simulink library "lib_TerCtrl_MASmsg"  (R2026a)
settings: Solver=VariableStepAuto
undefined symbols (not defined in the file): buses_lf, DiscIntNeverNeededParam, entity, iPs_lf, iQs_lf, last_send, m, Ps_lf, Qs_lf, Sb, set_asked, set_DG_up, set_extra_satur, set_sending_cost, v_buses_mod
libraries: simulink x581, sl_discontinuities x14, eeGeneralControl x7
(part 14 of 17)

== system lib_TerCtrl_MASmsg/MAS messages/ID6/Send to neighbor/four ==
  Message : Inport
  Cast1 : EntityMulticast  InputPortMessageModes=m  MulticastTag=ID1
  Cast1all : EntityMulticast  InputPortMessageModes=m  MulticastTag=ID1
  Cast2 : EntityMulticast  InputPortMessageModes=m  MulticastTag=ID3
  Cast2all : EntityMulticast  InputPortMessageModes=m  MulticastTag=ID3
  Cast3 : EntityMulticast  InputPortMessageModes=m  MulticastTag=ID0
  Cast3all : EntityMulticast  InputPortMessageModes=m  MulticastTag=ID0
  Cast4 : EntityMulticast  InputPortMessageModes=m  MulticastTag=ID0
  Cast4all : EntityMulticast  InputPortMessageModes=m  MulticastTag=ID0
  Entity Output Switch : EntityOutputSwitch  InputPortMessageModes=m  OutputPortMessageModes=m,m,m,m,m  NumberOutputPorts=5  SwitchingCriterion=From attribute  SwitchAttributeName=Select  InitialPortSelection=3
      settings: OutputPortMap=o0,o1,o2,o3,o4
  Entity Replicator1 : EntityReplicator  InputPortMessageModes=m  OutputPortMessageModes=m,m,m,m  NumberReplicas=3
      settings: OutputPortMap=o0,o1,o2,o3
  Entity Server : EntityServer  InputPortMessageModes=m  OutputPortMessageModes=m  Capacity=1  ServiceTimeValue=0  EntryAction=entity.Select = select(entity.Dest);
  select : Subsystem  TreatAsAtomicUnit=on
  wires:
  Entity Replicator1/3 -> Cast3all/1
  Entity Replicator1/4 -> Cast4all/1
  Entity Output Switch/5 -> Entity Replicator1/1
  Entity Output Switch/3 -> Cast3/1
  Entity Output Switch/1 -> Cast1/1
  Entity Replicator1/1 -> Cast1all/1
  Entity Replicator1/2 -> Cast2all/1
  Entity Output Switch/2 -> Cast2/1
  Entity Output Switch/4 -> Cast4/1
  Message/1 -> Entity Server/1  "Message"
  Entity Server/1 -> Entity Output Switch/1

== system lib_TerCtrl_MASmsg/MAS messages/ID6/Send to neighbor/one ==
  Message : Inport
  Cast : EntityMulticast  InputPortMessageModes=m  MulticastTag=ID2
  Castall : EntityMulticast  InputPortMessageModes=m  MulticastTag=ID2
  Entity Output Switch1 : EntityOutputSwitch  InputPortMessageModes=m  OutputPortMessageModes=m,m  SwitchingCriterion=From attribute  SwitchAttributeName=Select  InitialPortSelection=3
  Entity Server : EntityServer  InputPortMessageModes=m  OutputPortMessageModes=m  Capacity=1  ServiceTimeValue=0  EntryAction=entity.Select = select(entity.Dest);
  select : Subsystem  TreatAsAtomicUnit=on
  wires:
  Entity Output Switch1/2 -> Castall/1
  Entity Output Switch1/1 -> Cast/1
  Entity Server/1 -> Entity Output Switch1/1
  Message/1 -> Entity Server/1  "Message"

== system lib_TerCtrl_MASmsg/MAS messages/ID6/Send to neighbor/three ==
  Message : Inport
  Cast1 : EntityMulticast  InputPortMessageModes=m  MulticastTag=ID0
  Cast1all : EntityMulticast  InputPortMessageModes=m  MulticastTag=ID0
  Cast2 : EntityMulticast  InputPortMessageModes=m  MulticastTag=ID0
  Cast2all : EntityMulticast  InputPortMessageModes=m  MulticastTag=ID0
  Cast3 : EntityMulticast  InputPortMessageModes=m  MulticastTag=ID0
  Cast3all : EntityMulticast  InputPortMessageModes=m  MulticastTag=ID0
  Entity Output Switch : EntityOutputSwitch  InputPortMessageModes=m  OutputPortMessageModes=m,m,m,m  NumberOutputPorts=4  SwitchingCriterion=From attribute  SwitchAttributeName=Select  InitialPortSelection=3
      settings: OutputPortMap=o0,o1,o2,o3
  Entity Replicator1 : EntityReplicator  InputPortMessageModes=m  OutputPortMessageModes=m,m,m  NumberReplicas=2
      settings: OutputPortMap=o0,o1,o2
  Entity Server : EntityServer  InputPortMessageModes=m  OutputPortMessageModes=m  Capacity=1  ServiceTimeValue=0  EntryAction=entity.Select = select(entity.Dest);
  select : Subsystem  TreatAsAtomicUnit=on
  wires:
  Entity Output Switch/4 -> Entity Replicator1/1
  Entity Output Switch/2 -> Cast2/1
  Entity Replicator1/2 -> Cast2all/1
  Entity Replicator1/1 -> Cast1all/1
  Entity Output Switch/1 -> Cast1/1
  Entity Replicator1/3 -> Cast3all/1
  Entity Output Switch/3 -> Cast3/1
  Message/1 -> Entity Server/1  "Message"
  Entity Server/1 -> Entity Output Switch/1

== system lib_TerCtrl_MASmsg/MAS messages/ID6/Send to neighbor/two ==
  Message : Inport
  Cast1 : EntityMulticast  InputPortMessageModes=m  MulticastTag=ID5
  Cast1all : EntityMulticast  InputPortMessageModes=m  MulticastTag=ID5
  Cast2 : EntityMulticast  InputPortMessageModes=m  MulticastTag=ID7
  Cast2all : EntityMulticast  InputPortMessageModes=m  MulticastTag=ID7
  Entity Output Switch : EntityOutputSwitch  InputPortMessageModes=m  OutputPortMessageModes=m,m,m  NumberOutputPorts=3  SwitchingCriterion=From attribute  SwitchAttributeName=Select  InitialPortSelection=3
      settings: OutputPortMap=o0,o1,o2
  Entity Replicator1 : EntityReplicator  InputPortMessageModes=m  OutputPortMessageModes=m,m
  Entity Server : EntityServer  InputPortMessageModes=m  OutputPortMessageModes=m  Capacity=1  ServiceTimeValue=0  EntryAction=entity.Select = select(entity.Dest);
  select : Subsystem  TreatAsAtomicUnit=on
  wires:
  Entity Output Switch/3 -> Entity Replicator1/1
  Entity Replicator1/2 -> Cast2all/1
  Entity Replicator1/1 -> Cast1all/1
  Message/1 -> Entity Server/1  "Message"
  Entity Output Switch/1 -> Cast1/1
  Entity Output Switch/2 -> Cast2/1
  Entity Server/1 -> Entity Output Switch/1

== system lib_TerCtrl_MASmsg/MAS messages/ID6/Send to neighbor1/five ==
  Message : Inport
  Cast1 : EntityMulticast  InputPortMessageModes=m  MulticastTag=ID2
  Cast1all : EntityMulticast  InputPortMessageModes=m  MulticastTag=ID2
  Cast2 : EntityMulticast  InputPortMessageModes=m  MulticastTag=ID2
  Cast2all : EntityMulticast  InputPortMessageModes=m  MulticastTag=ID2
  Cast3 : EntityMulticast  InputPortMessageModes=m  MulticastTag=ID0
  Cast3all : EntityMulticast  InputPortMessageModes=m  MulticastTag=ID0
  Cast4 : EntityMulticast  InputPortMessageModes=m  MulticastTag=ID0
  Cast4all : EntityMulticast  InputPortMessageModes=m  MulticastTag=ID0
  Cast5 : EntityMulticast  InputPortMessageModes=m  MulticastTag=ID0
  Cast5all : EntityMulticast  InputPortMessageModes=m  MulticastTag=ID0
  Entity Output Switch : EntityOutputSwitch  InputPortMessageModes=m  OutputPortMessageModes=m,m,m,m,m,m  NumberOutputPorts=6  SwitchingCriterion=From attribute  SwitchAttributeName=Select  InitialPortSelection=3
      settings: OutputPortMap=o0,o1,o2,o3,o4,o5
  Entity Replicator1 : EntityReplicator  InputPortMessageModes=m  OutputPortMessageModes=m,m,m,m,m  NumberReplicas=4
      settings: OutputPortMap=o0,o1,o2,o3,o4
  Entity Server : EntityServer  InputPortMessageModes=m  OutputPortMessageModes=m  Capacity=1  ServiceTimeValue=0  EntryAction=entity.Select = select(entity.Dest);
  select : Subsystem  TreatAsAtomicUnit=on
  wires:
  Entity Server/1 -> Entity Output Switch/1
  Entity Output Switch/5 -> Cast5/1
  Entity Output Switch/1 -> Cast1/1
  Entity Replicator1/3 -> Cast3all/1
  Entity Replicator1/4 -> Cast4all/1
  Entity Output Switch/3 -> Cast3/1
  Entity Output Switch/2 -> Cast2/1
  Entity Replicator1/2 -> Cast2all/1
  Entity Replicator1/1 -> Cast1all/1
  Message/1 -> Entity Server/1  "Message"
  Entity Replicator1/5 -> Cast5all/1
  Entity Output Switch/6 -> Entity Replicator1/1
  Entity Output Switch/4 -> Cast4/1

== system lib_TerCtrl_MASmsg/MAS messages/ID6/Send to neighbor1/four ==
  Message : Inport
  Cast1 : EntityMulticast  InputPortMessageModes=m  MulticastTag=ID1
  Cast1all : EntityMulticast  InputPortMessageModes=m  MulticastTag=ID1
  Cast2 : EntityMulticast  InputPortMessageModes=m  MulticastTag=ID3
  Cast2all : EntityMulticast  InputPortMessageModes=m  MulticastTag=ID3
  Cast3 : EntityMulticast  InputPortMessageModes=m  MulticastTag=ID0
  Cast3all : EntityMulticast  InputPortMessageModes=m  MulticastTag=ID0
  Cast4 : EntityMulticast  InputPortMessageModes=m  MulticastTag=ID0
  Cast4all : EntityMulticast  InputPortMessageModes=m  MulticastTag=ID0
  Entity Output Switch : EntityOutputSwitch  InputPortMessageModes=m  OutputPortMessageModes=m,m,m,m,m  NumberOutputPorts=5  SwitchingCriterion=From attribute  SwitchAttributeName=Select  InitialPortSelection=3
      settings: OutputPortMap=o0,o1,o2,o3,o4
  Entity Replicator1 : EntityReplicator  InputPortMessageModes=m  OutputPortMessageModes=m,m,m,m  NumberReplicas=3
      settings: OutputPortMap=o0,o1,o2,o3
  Entity Server : EntityServer  InputPortMessageModes=m  OutputPortMessageModes=m  Capacity=1  ServiceTimeValue=0  EntryAction=entity.Select = select(entity.Dest);
  select : Subsystem  TreatAsAtomicUnit=on
  wires:
  Entity Server/1 -> Entity Output Switch/1
  Message/1 -> Entity Server/1  "Message"
  Entity Output Switch/4 -> Cast4/1
  Entity Output Switch/2 -> Cast2/1
  Entity Replicator1/2 -> Cast2all/1
  Entity Replicator1/1 -> Cast1all/1
  Entity Output Switch/1 -> Cast1/1
  Entity Output Switch/3 -> Cast3/1
  Entity Output Switch/5 -> Entity Replicator1/1
  Entity Replicator1/4 -> Cast4all/1
  Entity Replicator1/3 -> Cast3all/1

== system lib_TerCtrl_MASmsg/MAS messages/ID6/Send to neighbor1/one ==
  Message : Inport
  Cast : EntityMulticast  InputPortMessageModes=m  MulticastTag=ID2
  Castall : EntityMulticast  InputPortMessageModes=m  MulticastTag=ID2
  Entity Output Switch1 : EntityOutputSwitch  InputPortMessageModes=m  OutputPortMessageModes=m,m  SwitchingCriterion=From attribute  SwitchAttributeName=Select  InitialPortSelection=3
  Entity Server : EntityServer  InputPortMessageModes=m  OutputPortMessageModes=m  Capacity=1  ServiceTimeValue=0  EntryAction=entity.Select = select(entity.Dest);
  select : Subsystem  TreatAsAtomicUnit=on
  wires:
  Message/1 -> Entity Server/1  "Message"
  Entity Server/1 -> Entity Output Switch1/1
  Entity Output Switch1/1 -> Cast/1
  Entity Output Switch1/2 -> Castall/1

== system lib_TerCtrl_MASmsg/MAS messages/ID6/Send to neighbor1/three ==
  Message : Inport
  Cast1 : EntityMulticast  InputPortMessageModes=m  MulticastTag=ID0
  Cast1all : EntityMulticast  InputPortMessageModes=m  MulticastTag=ID0
  Cast2 : EntityMulticast  InputPortMessageModes=m  MulticastTag=ID0
  Cast2all : EntityMulticast  InputPortMessageModes=m  MulticastTag=ID0
  Cast3 : EntityMulticast  InputPortMessageModes=m  MulticastTag=ID0
  Cast3all : EntityMulticast  InputPortMessageModes=m  MulticastTag=ID0
  Entity Output Switch : EntityOutputSwitch  InputPortMessageModes=m  OutputPortMessageModes=m,m,m,m  NumberOutputPorts=4  SwitchingCriterion=From attribute  SwitchAttributeName=Select  InitialPortSelection=3
      settings: OutputPortMap=o0,o1,o2,o3
  Entity Replicator1 : EntityReplicator  InputPortMessageModes=m  OutputPortMessageModes=m,m,m  NumberReplicas=2
      settings: OutputPortMap=o0,o1,o2
  Entity Server : EntityServer  InputPortMessageModes=m  OutputPortMessageModes=m  Capacity=1  ServiceTimeValue=0  EntryAction=entity.Select = select(entity.Dest);
  select : Subsystem  TreatAsAtomicUnit=on
  wires:
  Entity Server/1 -> Entity Output Switch/1
  Message/1 -> Entity Server/1  "Message"
  Entity Output Switch/3 -> Cast3/1
  Entity Replicator1/3 -> Cast3all/1
  Entity Output Switch/1 -> Cast1/1
  Entity Replicator1/1 -> Cast1all/1
  Entity Replicator1/2 -> Cast2all/1
  Entity Output Switch/2 -> Cast2/1
  Entity Output Switch/4 -> Entity Replicator1/1

== system lib_TerCtrl_MASmsg/MAS messages/ID6/Send to neighbor1/two ==
  Message : Inport
  Cast1 : EntityMulticast  InputPortMessageModes=m  MulticastTag=ID5
  Cast1all : EntityMulticast  InputPortMessageModes=m  MulticastTag=ID5
  Cast2 : EntityMulticast  InputPortMessageModes=m  MulticastTag=ID7
  Cast2all : EntityMulticast  InputPortMessageModes=m  MulticastTag=ID7
  Entity Output Switch : EntityOutputSwitch  InputPortMessageModes=m  OutputPortMessageModes=m,m,m  NumberOutputPorts=3  SwitchingCriterion=From attribute  SwitchAttributeName=Select  InitialPortSelection=3
      settings: OutputPortMap=o0,o1,o2
  Entity Replicator1 : EntityReplicator  InputPortMessageModes=m  OutputPortMessageModes=m,m
  Entity Server : EntityServer  InputPortMessageModes=m  OutputPortMessageModes=m  Capacity=1  ServiceTimeValue=0  EntryAction=entity.Select = select(entity.Dest);
  select : Subsystem  TreatAsAtomicUnit=on
  wires:
  Entity Server/1 -> Entity Output Switch/1
  Entity Output Switch/2 -> Cast2/1
  Entity Output Switch/1 -> Cast1/1
  Message/1 -> Entity Server/1  "Message"
  Entity Replicator1/1 -> Cast1all/1
  Entity Replicator1/2 -> Cast2all/1
  Entity Output Switch/3 -> Entity Replicator1/1

== system lib_TerCtrl_MASmsg/MAS messages/ID6/Send to neighbor2/five ==
  Message : Inport
  Cast1 : EntityMulticast  InputPortMessageModes=m  MulticastTag=ID2
  Cast1all : EntityMulticast  InputPortMessageModes=m  MulticastTag=ID2
  Cast2 : EntityMulticast  InputPortMessageModes=m  MulticastTag=ID2
  Cast2all : EntityMulticast  InputPortMessageModes=m  MulticastTag=ID2
  Cast3 : EntityMulticast  InputPortMessageModes=m  MulticastTag=ID0
  Cast3all : EntityMulticast  InputPortMessageModes=m  MulticastTag=ID0
  Cast4 : EntityMulticast  InputPortMessageModes=m  MulticastTag=ID0
  Cast4all : EntityMulticast  InputPortMessageModes=m  MulticastTag=ID0
  Cast5 : EntityMulticast  InputPortMessageModes=m  MulticastTag=ID0
  Cast5all : EntityMulticast  InputPortMessageModes=m  MulticastTag=ID0
  Entity Output Switch : EntityOutputSwitch  InputPortMessageModes=m  OutputPortMessageModes=m,m,m,m,m,m  NumberOutputPorts=6  SwitchingCriterion=From attribute  SwitchAttributeName=Select  InitialPortSelection=3
      settings: OutputPortMap=o0,o1,o2,o3,o4,o5
  Entity Replicator1 : EntityReplicator  InputPortMessageModes=m  OutputPortMessageModes=m,m,m,m,m  NumberReplicas=4
      settings: OutputPortMap=o0,o1,o2,o3,o4
  Entity Server : EntityServer  InputPortMessageModes=m  OutputPortMessageModes=m  Capacity=1  ServiceTimeValue=0  EntryAction=entity.Select = select(entity.Dest);
  select : Subsystem  TreatAsAtomicUnit=on
  wires:
  Entity Output Switch/4 -> Cast4/1
  Entity Output Switch/6 -> Entity Replicator1/1
  Entity Replicator1/5 -> Cast5all/1
  Message/1 -> Entity Server/1  "Message"
  Entity Replicator1/1 -> Cast1all/1
  Entity Replicator1/2 -> Cast2all/1
  Entity Output Switch/2 -> Cast2/1
  Entity Output Switch/3 -> Cast3/1
  Entity Replicator1/4 -> Cast4all/1
  Entity Replicator1/3 -> Cast3all/1
  Entity Output Switch/1 -> Cast1/1
  Entity Output Switch/5 -> Cast5/1
  Entity Server/1 -> Entity Output Switch/1

== system lib_TerCtrl_MASmsg/MAS messages/ID6/Send to neighbor2/four ==
  Message : Inport
  Cast1 : EntityMulticast  InputPortMessageModes=m  MulticastTag=ID1
  Cast1all : EntityMulticast  InputPortMessageModes=m  MulticastTag=ID1
  Cast2 : EntityMulticast  InputPortMessageModes=m  MulticastTag=ID3
  Cast2all : EntityMulticast  InputPortMessageModes=m  MulticastTag=ID3
  Cast3 : EntityMulticast  InputPortMessageModes=m  MulticastTag=ID0
  Cast3all : EntityMulticast  InputPortMessageModes=m  MulticastTag=ID0
  Cast4 : EntityMulticast  InputPortMessageModes=m  MulticastTag=ID0
  Cast4all : EntityMulticast  InputPortMessageModes=m  MulticastTag=ID0
  Entity Output Switch : EntityOutputSwitch  InputPortMessageModes=m  OutputPortMessageModes=m,m,m,m,m  NumberOutputPorts=5  SwitchingCriterion=From attribute  SwitchAttributeName=Select  InitialPortSelection=3
      settings: OutputPortMap=o0,o1,o2,o3,o4
  Entity Replicator1 : EntityReplicator  InputPortMessageModes=m  OutputPortMessageModes=m,m,m,m  NumberReplicas=3
      settings: OutputPortMap=o0,o1,o2,o3
  Entity Server : EntityServer  InputPortMessageModes=m  OutputPortMessageModes=m  Capacity=1  ServiceTimeValue=0  EntryAction=entity.Select = select(entity.Dest);
  select : Subsystem  TreatAsAtomicUnit=on
  wires:
  Entity Replicator1/3 -> Cast3all/1
  Entity Replicator1/4 -> Cast4all/1
  Entity Output Switch/5 -> Entity Replicator1/1
  Entity Output Switch/3 -> Cast3/1
  Entity Output Switch/1 -> Cast1/1
  Entity Replicator1/1 -> Cast1all/1
  Entity Replicator1/2 -> Cast2all/1
  Entity Output Switch/2 -> Cast2/1
  Entity Output Switch/4 -> Cast4/1
  Message/1 -> Entity Server/1  "Message"
  Entity Server/1 -> Entity Output Switch/1

== system lib_TerCtrl_MASmsg/MAS messages/ID6/Send to neighbor2/one ==
  Message : Inport
  Cast : EntityMulticast  InputPortMessageModes=m  MulticastTag=ID2
  Castall : EntityMulticast  InputPortMessageModes=m  MulticastTag=ID2
  Entity Output Switch1 : EntityOutputSwitch  InputPortMessageModes=m  OutputPortMessageModes=m,m  SwitchingCriterion=From attribute  SwitchAttributeName=Select  InitialPortSelection=3
  Entity Server : EntityServer  InputPortMessageModes=m  OutputPortMessageModes=m  Capacity=1  ServiceTimeValue=0  EntryAction=entity.Select = select(entity.Dest);
  select : Subsystem  TreatAsAtomicUnit=on
  wires:
  Entity Output Switch1/2 -> Castall/1
  Entity Output Switch1/1 -> Cast/1
  Entity Server/1 -> Entity Output Switch1/1
  Message/1 -> Entity Server/1  "Message"

== system lib_TerCtrl_MASmsg/MAS messages/ID6/Send to neighbor2/three ==
  Message : Inport
  Cast1 : EntityMulticast  InputPortMessageModes=m  MulticastTag=ID0
  Cast1all : EntityMulticast  InputPortMessageModes=m  MulticastTag=ID0
  Cast2 : EntityMulticast  InputPortMessageModes=m  MulticastTag=ID0
  Cast2all : EntityMulticast  InputPortMessageModes=m  MulticastTag=ID0
  Cast3 : EntityMulticast  InputPortMessageModes=m  MulticastTag=ID0
  Cast3all : EntityMulticast  InputPortMessageModes=m  MulticastTag=ID0
  Entity Output Switch : EntityOutputSwitch  InputPortMessageModes=m  OutputPortMessageModes=m,m,m,m  NumberOutputPorts=4  SwitchingCriterion=From attribute  SwitchAttributeName=Select  InitialPortSelection=3
      settings: OutputPortMap=o0,o1,o2,o3
  Entity Replicator1 : EntityReplicator  InputPortMessageModes=m  OutputPortMessageModes=m,m,m  NumberReplicas=2
      settings: OutputPortMap=o0,o1,o2
  Entity Server : EntityServer  InputPortMessageModes=m  OutputPortMessageModes=m  Capacity=1  ServiceTimeValue=0  EntryAction=entity.Select = select(entity.Dest);
  select : Subsystem  TreatAsAtomicUnit=on
  wires:
  Entity Output Switch/4 -> Entity Replicator1/1
  Entity Output Switch/2 -> Cast2/1
  Entity Replicator1/2 -> Cast2all/1
  Entity Replicator1/1 -> Cast1all/1
  Entity Output Switch/1 -> Cast1/1
  Entity Replicator1/3 -> Cast3all/1
  Entity Output Switch/3 -> Cast3/1
  Message/1 -> Entity Server/1  "Message"
  Entity Server/1 -> Entity Output Switch/1

== system lib_TerCtrl_MASmsg/MAS messages/ID6/Send to neighbor2/two ==
  Message : Inport
  Cast1 : EntityMulticast  InputPortMessageModes=m  MulticastTag=ID5
  Cast1all : EntityMulticast  InputPortMessageModes=m  MulticastTag=ID5
  Cast2 : EntityMulticast  InputPortMessageModes=m  MulticastTag=ID7
  Cast2all : EntityMulticast  InputPortMessageModes=m  MulticastTag=ID7
  Entity Output Switch : EntityOutputSwitch  InputPortMessageModes=m  OutputPortMessageModes=m,m,m  NumberOutputPorts=3  SwitchingCriterion=From attribute  SwitchAttributeName=Select  InitialPortSelection=3
      settings: OutputPortMap=o0,o1,o2
  Entity Replicator1 : EntityReplicator  InputPortMessageModes=m  OutputPortMessageModes=m,m
  Entity Server : EntityServer  InputPortMessageModes=m  OutputPortMessageModes=m  Capacity=1  ServiceTimeValue=0  EntryAction=entity.Select = select(entity.Dest);
  select : Subsystem  TreatAsAtomicUnit=on
  wires:
  Entity Output Switch/3 -> Entity Replicator1/1
  Entity Replicator1/2 -> Cast2all/1
  Entity Replicator1/1 -> Cast1all/1
  Message/1 -> Entity Server/1  "Message"
  Entity Output Switch/1 -> Cast1/1
  Entity Output Switch/2 -> Cast2/1
  Entity Server/1 -> Entity Output Switch/1

== system lib_TerCtrl_MASmsg/MAS messages/ID7/Send to neighbor/five ==
  Message : Inport
  Cast1 : EntityMulticast  InputPortMessageModes=m  MulticastTag=ID2
  Cast1all : EntityMulticast  InputPortMessageModes=m  MulticastTag=ID2
  Cast2 : EntityMulticast  InputPortMessageModes=m  MulticastTag=ID2
  Cast2all : EntityMulticast  InputPortMessageModes=m  MulticastTag=ID2
  Cast3 : EntityMulticast  InputPortMessageModes=m  MulticastTag=ID0
  Cast3all : EntityMulticast  InputPortMessageModes=m  MulticastTag=ID0
  Cast4 : EntityMulticast  InputPortMessageModes=m  MulticastTag=ID0
  Cast4all : EntityMulticast  InputPortMessageModes=m  MulticastTag=ID0
  Cast5 : EntityMulticast  InputPortMessageModes=m  MulticastTag=ID0
  Cast5all : EntityMulticast  InputPortMessageModes=m  MulticastTag=ID0
  Entity Output Switch : EntityOutputSwitch  InputPortMessageModes=m  OutputPortMessageModes=m,m,m,m,m,m  NumberOutputPorts=6  SwitchingCriterion=From attribute  SwitchAttributeName=Select  InitialPortSelection=3
      settings: OutputPortMap=o0,o1,o2,o3,o4,o5
  Entity Replicator1 : EntityReplicator  InputPortMessageModes=m  OutputPortMessageModes=m,m,m,m,m  NumberReplicas=4
      settings: OutputPortMap=o0,o1,o2,o3,o4
  Entity Server : EntityServer  InputPortMessageModes=m  OutputPortMessageModes=m  Capacity=1  ServiceTimeValue=0  EntryAction=entity.Select = select(entity.Dest);
  select : Subsystem  TreatAsAtomicUnit=on
  wires:
  Entity Output Switch/4 -> Cast4/1
  Entity Output Switch/6 -> Entity Replicator1/1
  Entity Replicator1/5 -> Cast5all/1
  Message/1 -> Entity Server/1  "Message"
  Entity Replicator1/1 -> Cast1all/1
  Entity Replicator1/2 -> Cast2all/1
  Entity Output Switch/2 -> Cast2/1
  Entity Output Switch/3 -> Cast3/1
  Entity Replicator1/4 -> Cast4all/1
  Entity Replicator1/3 -> Cast3all/1
  Entity Output Switch/1 -> Cast1/1
  Entity Output Switch/5 -> Cast5/1
  Entity Server/1 -> Entity Output Switch/1

== system lib_TerCtrl_MASmsg/MAS messages/ID7/Send to neighbor/four ==
  Message : Inport
  Cast1 : EntityMulticast  InputPortMessageModes=m  MulticastTag=ID1
  Cast1all : EntityMulticast  InputPortMessageModes=m  MulticastTag=ID1
  Cast2 : EntityMulticast  InputPortMessageModes=m  MulticastTag=ID3
  Cast2all : EntityMulticast  InputPortMessageModes=m  MulticastTag=ID3
  Cast3 : EntityMulticast  InputPortMessageModes=m  MulticastTag=ID0
  Cast3all : EntityMulticast  InputPortMessageModes=m  MulticastTag=ID0
  Cast4 : EntityMulticast  InputPortMessageModes=m  MulticastTag=ID0
  Cast4all : EntityMulticast  InputPortMessageModes=m  MulticastTag=ID0
  Entity Output Switch : EntityOutputSwitch  InputPortMessageModes=m  OutputPortMessageModes=m,m,m,m,m  NumberOutputPorts=5  SwitchingCriterion=From attribute  SwitchAttributeName=Select  InitialPortSelection=3
      settings: OutputPortMap=o0,o1,o2,o3,o4
  Entity Replicator1 : EntityReplicator  InputPortMessageModes=m  OutputPortMessageModes=m,m,m,m  NumberReplicas=3
      settings: OutputPortMap=o0,o1,o2,o3
  Entity Server : EntityServer  InputPortMessageModes=m  OutputPortMessageModes=m  Capacity=1  ServiceTimeValue=0  EntryAction=entity.Select = select(entity.Dest);
  select : Subsystem  TreatAsAtomicUnit=on
  wires:
  Entity Replicator1/3 -> Cast3all/1
  Entity Replicator1/4 -> Cast4all/1
  Entity Output Switch/5 -> Entity Replicator1/1
  Entity Output Switch/3 -> Cast3/1
  Entity Output Switch/1 -> Cast1/1
  Entity Replicator1/1 -> Cast1all/1
  Entity Replicator1/2 -> Cast2all/1
  Entity Output Switch/2 -> Cast2/1
  Entity Output Switch/4 -> Cast4/1
  Message/1 -> Entity Server/1  "Message"
  Entity Server/1 -> Entity Output Switch/1

== system lib_TerCtrl_MASmsg/MAS messages/ID7/Send to neighbor/one ==
  Message : Inport
  Cast : EntityMulticast  InputPortMessageModes=m  MulticastTag=ID2
  Castall : EntityMulticast  InputPortMessageModes=m  MulticastTag=ID2
  Entity Output Switch1 : EntityOutputSwitch  InputPortMessageModes=m  OutputPortMessageModes=m,m  SwitchingCriterion=From attribute  SwitchAttributeName=Select  InitialPortSelection=3
  Entity Server : EntityServer  InputPortMessageModes=m  OutputPortMessageModes=m  Capacity=1  ServiceTimeValue=0  EntryAction=entity.Select = select(entity.Dest);
  select : Subsystem  TreatAsAtomicUnit=on
  wires:
  Entity Output Switch1/2 -> Castall/1
  Entity Output Switch1/1 -> Cast/1
  Entity Server/1 -> Entity Output Switch1/1
  Message/1 -> Entity Server/1  "Message"

== system lib_TerCtrl_MASmsg/MAS messages/ID7/Send to neighbor/three ==
  Message : Inport
  Cast1 : EntityMulticast  InputPortMessageModes=m  MulticastTag=ID0
  Cast1all : EntityMulticast  InputPortMessageModes=m  MulticastTag=ID0
  Cast2 : EntityMulticast  InputPortMessageModes=m  MulticastTag=ID0
  Cast2all : EntityMulticast  InputPortMessageModes=m  MulticastTag=ID0
  Cast3 : EntityMulticast  InputPortMessageModes=m  MulticastTag=ID0
  Cast3all : EntityMulticast  InputPortMessageModes=m  MulticastTag=ID0
  Entity Output Switch : EntityOutputSwitch  InputPortMessageModes=m  OutputPortMessageModes=m,m,m,m  NumberOutputPorts=4  SwitchingCriterion=From attribute  SwitchAttributeName=Select  InitialPortSelection=3
      settings: OutputPortMap=o0,o1,o2,o3
  Entity Replicator1 : EntityReplicator  InputPortMessageModes=m  OutputPortMessageModes=m,m,m  NumberReplicas=2
      settings: OutputPortMap=o0,o1,o2
  Entity Server : EntityServer  InputPortMessageModes=m  OutputPortMessageModes=m  Capacity=1  ServiceTimeValue=0  EntryAction=entity.Select = select(entity.Dest);
  select : Subsystem  TreatAsAtomicUnit=on
  wires:
  Entity Output Switch/4 -> Entity Replicator1/1
  Entity Output Switch/2 -> Cast2/1
  Entity Replicator1/2 -> Cast2all/1
  Entity Replicator1/1 -> Cast1all/1
  Entity Output Switch/1 -> Cast1/1
  Entity Replicator1/3 -> Cast3all/1
  Entity Output Switch/3 -> Cast3/1
  Message/1 -> Entity Server/1  "Message"
  Entity Server/1 -> Entity Output Switch/1

== system lib_TerCtrl_MASmsg/MAS messages/ID7/Send to neighbor/two ==
  Message : Inport
  Cast1 : EntityMulticast  InputPortMessageModes=m  MulticastTag=ID6
  Cast1all : EntityMulticast  InputPortMessageModes=m  MulticastTag=ID6
  Cast2 : EntityMulticast  InputPortMessageModes=m  MulticastTag=ID1
  Cast2all : EntityMulticast  InputPortMessageModes=m  MulticastTag=ID1
  Entity Output Switch : EntityOutputSwitch  InputPortMessageModes=m  OutputPortMessageModes=m,m,m  NumberOutputPorts=3  SwitchingCriterion=From attribute  SwitchAttributeName=Select  InitialPortSelection=3
      settings: OutputPortMap=o0,o1,o2
  Entity Replicator1 : EntityReplicator  InputPortMessageModes=m  OutputPortMessageModes=m,m
  Entity Server : EntityServer  InputPortMessageModes=m  OutputPortMessageModes=m  Capacity=1  ServiceTimeValue=0  EntryAction=entity.Select = select(entity.Dest);
  select : Subsystem  TreatAsAtomicUnit=on
  wires:
  Entity Output Switch/3 -> Entity Replicator1/1
  Entity Replicator1/2 -> Cast2all/1
  Entity Replicator1/1 -> Cast1all/1
  Message/1 -> Entity Server/1  "Message"
  Entity Output Switch/1 -> Cast1/1
  Entity Output Switch/2 -> Cast2/1
  Entity Server/1 -> Entity Output Switch/1

== system lib_TerCtrl_MASmsg/MAS messages/ID7/Send to neighbor1/five ==
  Message : Inport
  Cast1 : EntityMulticast  InputPortMessageModes=m  MulticastTag=ID2
  Cast1all : EntityMulticast  InputPortMessageModes=m  MulticastTag=ID2
  Cast2 : EntityMulticast  InputPortMessageModes=m  MulticastTag=ID2
  Cast2all : EntityMulticast  InputPortMessageModes=m  MulticastTag=ID2
  Cast3 : EntityMulticast  InputPortMessageModes=m  MulticastTag=ID0
  Cast3all : EntityMulticast  InputPortMessageModes=m  MulticastTag=ID0
  Cast4 : EntityMulticast  InputPortMessageModes=m  MulticastTag=ID0
  Cast4all : EntityMulticast  InputPortMessageModes=m  MulticastTag=ID0
  Cast5 : EntityMulticast  InputPortMessageModes=m  MulticastTag=ID0
  Cast5all : EntityMulticast  InputPortMessageModes=m  MulticastTag=ID0
  Entity Output Switch : EntityOutputSwitch  InputPortMessageModes=m  OutputPortMessageModes=m,m,m,m,m,m  NumberOutputPorts=6  SwitchingCriterion=From attribute  SwitchAttributeName=Select  InitialPortSelection=3
      settings: OutputPortMap=o0,o1,o2,o3,o4,o5
  Entity Replicator1 : EntityReplicator  InputPortMessageModes=m  OutputPortMessageModes=m,m,m,m,m  NumberReplicas=4
      settings: OutputPortMap=o0,o1,o2,o3,o4
  Entity Server : EntityServer  InputPortMessageModes=m  OutputPortMessageModes=m  Capacity=1  ServiceTimeValue=0  EntryAction=entity.Select = select(entity.Dest);
  select : Subsystem  TreatAsAtomicUnit=on
  wires:
  Entity Server/1 -> Entity Output Switch/1
  Entity Output Switch/5 -> Cast5/1
  Entity Output Switch/1 -> Cast1/1
  Entity Replicator1/3 -> Cast3all/1
  Entity Replicator1/4 -> Cast4all/1
  Entity Output Switch/3 -> Cast3/1
  Entity Output Switch/2 -> Cast2/1
  Entity Replicator1/2 -> Cast2all/1
  Entity Replicator1/1 -> Cast1all/1
  Message/1 -> Entity Server/1  "Message"
  Entity Replicator1/5 -> Cast5all/1
  Entity Output Switch/6 -> Entity Replicator1/1
  Entity Output Switch/4 -> Cast4/1

== system lib_TerCtrl_MASmsg/MAS messages/ID7/Send to neighbor1/four ==
  Message : Inport
  Cast1 : EntityMulticast  InputPortMessageModes=m  MulticastTag=ID1
  Cast1all : EntityMulticast  InputPortMessageModes=m  MulticastTag=ID1
  Cast2 : EntityMulticast  InputPortMessageModes=m  MulticastTag=ID3
  Cast2all : EntityMulticast  InputPortMessageModes=m  MulticastTag=ID3
  Cast3 : EntityMulticast  InputPortMessageModes=m  MulticastTag=ID0
  Cast3all : EntityMulticast  InputPortMessageModes=m  MulticastTag=ID0
  Cast4 : EntityMulticast  InputPortMessageModes=m  MulticastTag=ID0
  Cast4all : EntityMulticast  InputPortMessageModes=m  MulticastTag=ID0
  Entity Output Switch : EntityOutputSwitch  InputPortMessageModes=m  OutputPortMessageModes=m,m,m,m,m  NumberOutputPorts=5  SwitchingCriterion=From attribute  SwitchAttributeName=Select  InitialPortSelection=3
      settings: OutputPortMap=o0,o1,o2,o3,o4
  Entity Replicator1 : EntityReplicator  InputPortMessageModes=m  OutputPortMessageModes=m,m,m,m  NumberReplicas=3
      settings: OutputPortMap=o0,o1,o2,o3
  Entity Server : EntityServer  InputPortMessageModes=m  OutputPortMessageModes=m  Capacity=1  ServiceTimeValue=0  EntryAction=entity.Select = select(entity.Dest);
  select : Subsystem  TreatAsAtomicUnit=on
  wires:
  Entity Server/1 -> Entity Output Switch/1
  Message/1 -> Entity Server/1  "Message"
  Entity Output Switch/4 -> Cast4/1
  Entity Output Switch/2 -> Cast2/1
  Entity Replicator1/2 -> Cast2all/1
  Entity Replicator1/1 -> Cast1all/1
  Entity Output Switch/1 -> Cast1/1
  Entity Output Switch/3 -> Cast3/1
  Entity Output Switch/5 -> Entity Replicator1/1
  Entity Replicator1/4 -> Cast4all/1
  Entity Replicator1/3 -> Cast3all/1

== system lib_TerCtrl_MASmsg/MAS messages/ID7/Send to neighbor1/one ==
  Message : Inport
  Cast : EntityMulticast  InputPortMessageModes=m  MulticastTag=ID2
  Castall : EntityMulticast  InputPortMessageModes=m  MulticastTag=ID2
  Entity Output Switch1 : EntityOutputSwitch  InputPortMessageModes=m  OutputPortMessageModes=m,m  SwitchingCriterion=From attribute  SwitchAttributeName=Select  InitialPortSelection=3
  Entity Server : EntityServer  InputPortMessageModes=m  OutputPortMessageModes=m  Capacity=1  ServiceTimeValue=0  EntryAction=entity.Select = select(entity.Dest);
  select : Subsystem  TreatAsAtomicUnit=on
  wires:
  Message/1 -> Entity Server/1  "Message"
  Entity Server/1 -> Entity Output Switch1/1
  Entity Output Switch1/1 -> Cast/1
  Entity Output Switch1/2 -> Castall/1

== system lib_TerCtrl_MASmsg/MAS messages/ID7/Send to neighbor1/three ==
  Message : Inport
  Cast1 : EntityMulticast  InputPortMessageModes=m  MulticastTag=ID0
  Cast1all : EntityMulticast  InputPortMessageModes=m  MulticastTag=ID0
  Cast2 : EntityMulticast  InputPortMessageModes=m  MulticastTag=ID0
  Cast2all : EntityMulticast  InputPortMessageModes=m  MulticastTag=ID0
  Cast3 : EntityMulticast  InputPortMessageModes=m  MulticastTag=ID0
  Cast3all : EntityMulticast  InputPortMessageModes=m  MulticastTag=ID0
  Entity Output Switch : EntityOutputSwitch  InputPortMessageModes=m  OutputPortMessageModes=m,m,m,m  NumberOutputPorts=4  SwitchingCriterion=From attribute  SwitchAttributeName=Select  InitialPortSelection=3
      settings: OutputPortMap=o0,o1,o2,o3
  Entity Replicator1 : EntityReplicator  InputPortMessageModes=m  OutputPortMessageModes=m,m,m  NumberReplicas=2
      settings: OutputPortMap=o0,o1,o2
  Entity Server : EntityServer  InputPortMessageModes=m  OutputPortMessageModes=m  Capacity=1  ServiceTimeValue=0  EntryAction=entity.Select = select(entity.Dest);
  select : Subsystem  TreatAsAtomicUnit=on
  wires:
  Entity Server/1 -> Entity Output Switch/1
  Message/1 -> Entity Server/1  "Message"
  Entity Output Switch/3 -> Cast3/1
  Entity Replicator1/3 -> Cast3all/1
  Entity Output Switch/1 -> Cast1/1
  Entity Replicator1/1 -> Cast1all/1
  Entity Replicator1/2 -> Cast2all/1
  Entity Output Switch/2 -> Cast2/1
  Entity Output Switch/4 -> Entity Replicator1/1

== system lib_TerCtrl_MASmsg/MAS messages/ID7/Send to neighbor1/two ==
  Message : Inport
  Cast1 : EntityMulticast  InputPortMessageModes=m  MulticastTag=ID6
  Cast1all : EntityMulticast  InputPortMessageModes=m  MulticastTag=ID6
  Cast2 : EntityMulticast  InputPortMessageModes=m  MulticastTag=ID1
  Cast2all : EntityMulticast  InputPortMessageModes=m  MulticastTag=ID1
  Entity Output Switch : EntityOutputSwitch  InputPortMessageModes=m  OutputPortMessageModes=m,m,m  NumberOutputPorts=3  SwitchingCriterion=From attribute  SwitchAttributeName=Select  InitialPortSelection=3
      settings: OutputPortMap=o0,o1,o2
  Entity Replicator1 : EntityReplicator  InputPortMessageModes=m  OutputPortMessageModes=m,m
  Entity Server : EntityServer  InputPortMessageModes=m  OutputPortMessageModes=m  Capacity=1  ServiceTimeValue=0  EntryAction=entity.Select = select(entity.Dest);
  select : Subsystem  TreatAsAtomicUnit=on
  wires:
  Entity Server/1 -> Entity Output Switch/1
  Entity Output Switch/2 -> Cast2/1
  Entity Output Switch/1 -> Cast1/1
  Message/1 -> Entity Server/1  "Message"
  Entity Replicator1/1 -> Cast1all/1
  Entity Replicator1/2 -> Cast2all/1
  Entity Output Switch/3 -> Entity Replicator1/1

== system lib_TerCtrl_MASmsg/MAS messages/ID7/Send to neighbor2/five ==
  Message : Inport
  Cast1 : EntityMulticast  InputPortMessageModes=m  MulticastTag=ID2
  Cast1all : EntityMulticast  InputPortMessageModes=m  MulticastTag=ID2
  Cast2 : EntityMulticast  InputPortMessageModes=m  MulticastTag=ID2
  Cast2all : EntityMulticast  InputPortMessageModes=m  MulticastTag=ID2
  Cast3 : EntityMulticast  InputPortMessageModes=m  MulticastTag=ID0
  Cast3all : EntityMulticast  InputPortMessageModes=m  MulticastTag=ID0
  Cast4 : EntityMulticast  InputPortMessageModes=m  MulticastTag=ID0
  Cast4all : EntityMulticast  InputPortMessageModes=m  MulticastTag=ID0
  Cast5 : EntityMulticast  InputPortMessageModes=m  MulticastTag=ID0
  Cast5all : EntityMulticast  InputPortMessageModes=m  MulticastTag=ID0
  Entity Output Switch : EntityOutputSwitch  InputPortMessageModes=m  OutputPortMessageModes=m,m,m,m,m,m  NumberOutputPorts=6  SwitchingCriterion=From attribute  SwitchAttributeName=Select  InitialPortSelection=3
      settings: OutputPortMap=o0,o1,o2,o3,o4,o5
  Entity Replicator1 : EntityReplicator  InputPortMessageModes=m  OutputPortMessageModes=m,m,m,m,m  NumberReplicas=4
      settings: OutputPortMap=o0,o1,o2,o3,o4
  Entity Server : EntityServer  InputPortMessageModes=m  OutputPortMessageModes=m  Capacity=1  ServiceTimeValue=0  EntryAction=entity.Select = select(entity.Dest);
  select : Subsystem  TreatAsAtomicUnit=on
  wires:
  Entity Output Switch/4 -> Cast4/1
  Entity Output Switch/6 -> Entity Replicator1/1
  Entity Replicator1/5 -> Cast5all/1
  Message/1 -> Entity Server/1  "Message"
  Entity Replicator1/1 -> Cast1all/1
  Entity Replicator1/2 -> Cast2all/1
  Entity Output Switch/2 -> Cast2/1
  Entity Output Switch/3 -> Cast3/1
  Entity Replicator1/4 -> Cast4all/1
  Entity Replicator1/3 -> Cast3all/1
  Entity Output Switch/1 -> Cast1/1
  Entity Output Switch/5 -> Cast5/1
  Entity Server/1 -> Entity Output Switch/1

== system lib_TerCtrl_MASmsg/MAS messages/ID7/Send to neighbor2/four ==
  Message : Inport
  Cast1 : EntityMulticast  InputPortMessageModes=m  MulticastTag=ID1
  Cast1all : EntityMulticast  InputPortMessageModes=m  MulticastTag=ID1
  Cast2 : EntityMulticast  InputPortMessageModes=m  MulticastTag=ID3
  Cast2all : EntityMulticast  InputPortMessageModes=m  MulticastTag=ID3
  Cast3 : EntityMulticast  InputPortMessageModes=m  MulticastTag=ID0
  Cast3all : EntityMulticast  InputPortMessageModes=m  MulticastTag=ID0
  Cast4 : EntityMulticast  InputPortMessageModes=m  MulticastTag=ID0
  Cast4all : EntityMulticast  InputPortMessageModes=m  MulticastTag=ID0
  Entity Output Switch : EntityOutputSwitch  InputPortMessageModes=m  OutputPortMessageModes=m,m,m,m,m  NumberOutputPorts=5  SwitchingCriterion=From attribute  SwitchAttributeName=Select  InitialPortSelection=3
      settings: OutputPortMap=o0,o1,o2,o3,o4
  Entity Replicator1 : EntityReplicator  InputPortMessageModes=m  OutputPortMessageModes=m,m,m,m  NumberReplicas=3
      settings: OutputPortMap=o0,o1,o2,o3
  Entity Server : EntityServer  InputPortMessageModes=m  OutputPortMessageModes=m  Capacity=1  ServiceTimeValue=0  EntryAction=entity.Select = select(entity.Dest);
  select : Subsystem  TreatAsAtomicUnit=on
  wires:
  Entity Replicator1/3 -> Cast3all/1
  Entity Replicator1/4 -> Cast4all/1
  Entity Output Switch/5 -> Entity Replicator1/1
  Entity Output Switch/3 -> Cast3/1
  Entity Output Switch/1 -> Cast1/1
  Entity Replicator1/1 -> Cast1all/1
  Entity Replicator1/2 -> Cast2all/1
  Entity Output Switch/2 -> Cast2/1
  Entity Output Switch/4 -> Cast4/1
  Message/1 -> Entity Server/1  "Message"
  Entity Server/1 -> Entity Output Switch/1

== system lib_TerCtrl_MASmsg/MAS messages/ID7/Send to neighbor2/one ==
  Message : Inport
  Cast : EntityMulticast  InputPortMessageModes=m  MulticastTag=ID2
  Castall : EntityMulticast  InputPortMessageModes=m  MulticastTag=ID2
  Entity Output Switch1 : EntityOutputSwitch  InputPortMessageModes=m  OutputPortMessageModes=m,m  SwitchingCriterion=From attribute  SwitchAttributeName=Select  InitialPortSelection=3
  Entity Server : EntityServer  InputPortMessageModes=m  OutputPortMessageModes=m  Capacity=1  ServiceTimeValue=0  EntryAction=entity.Select = select(entity.Dest);
  select : Subsystem  TreatAsAtomicUnit=on
  wires:
  Entity Output Switch1/2 -> Castall/1
  Entity Output Switch1/1 -> Cast/1
  Entity Server/1 -> Entity Output Switch1/1
  Message/1 -> Entity Server/1  "Message"

== system lib_TerCtrl_MASmsg/MAS messages/ID7/Send to neighbor2/three ==
  Message : Inport
  Cast1 : EntityMulticast  InputPortMessageModes=m  MulticastTag=ID0
  Cast1all : EntityMulticast  InputPortMessageModes=m  MulticastTag=ID0
  Cast2 : EntityMulticast  InputPortMessageModes=m  MulticastTag=ID0
  Cast2all : EntityMulticast  InputPortMessageModes=m  MulticastTag=ID0
  Cast3 : EntityMulticast  InputPortMessageModes=m  MulticastTag=ID0
  Cast3all : EntityMulticast  InputPortMessageModes=m  MulticastTag=ID0
  Entity Output Switch : EntityOutputSwitch  InputPortMessageModes=m  OutputPortMessageModes=m,m,m,m  NumberOutputPorts=4  SwitchingCriterion=From attribute  SwitchAttributeName=Select  InitialPortSelection=3
      settings: OutputPortMap=o0,o1,o2,o3
  Entity Replicator1 : EntityReplicator  InputPortMessageModes=m  OutputPortMessageModes=m,m,m  NumberReplicas=2
      settings: OutputPortMap=o0,o1,o2
  Entity Server : EntityServer  InputPortMessageModes=m  OutputPortMessageModes=m  Capacity=1  ServiceTimeValue=0  EntryAction=entity.Select = select(entity.Dest);
  select : Subsystem  TreatAsAtomicUnit=on
  wires:
  Entity Output Switch/4 -> Entity Replicator1/1
  Entity Output Switch/2 -> Cast2/1
  Entity Replicator1/2 -> Cast2all/1
  Entity Replicator1/1 -> Cast1all/1
  Entity Output Switch/1 -> Cast1/1
  Entity Replicator1/3 -> Cast3all/1
  Entity Output Switch/3 -> Cast3/1
  Message/1 -> Entity Server/1  "Message"
  Entity Server/1 -> Entity Output Switch/1

== system lib_TerCtrl_MASmsg/MAS messages/ID7/Send to neighbor2/two ==
  Message : Inport
  Cast1 : EntityMulticast  InputPortMessageModes=m  MulticastTag=ID6
  Cast1all : EntityMulticast  InputPortMessageModes=m  MulticastTag=ID6
  Cast2 : EntityMulticast  InputPortMessageModes=m  MulticastTag=ID1
  Cast2all : EntityMulticast  InputPortMessageModes=m  MulticastTag=ID1
  Entity Output Switch : EntityOutputSwitch  InputPortMessageModes=m  OutputPortMessageModes=m,m,m  NumberOutputPorts=3  SwitchingCriterion=From attribute  SwitchAttributeName=Select  InitialPortSelection=3
      settings: OutputPortMap=o0,o1,o2
  Entity Replicator1 : EntityReplicator  InputPortMessageModes=m  OutputPortMessageModes=m,m
  Entity Server : EntityServer  InputPortMessageModes=m  OutputPortMessageModes=m  Capacity=1  ServiceTimeValue=0  EntryAction=entity.Select = select(entity.Dest);
  select : Subsystem  TreatAsAtomicUnit=on
  wires:
  Entity Output Switch/3 -> Entity Replicator1/1
  Entity Replicator1/2 -> Cast2all/1
  Entity Replicator1/1 -> Cast1all/1
  Message/1 -> Entity Server/1  "Message"
  Entity Output Switch/1 -> Cast1/1
  Entity Output Switch/2 -> Cast2/1
  Entity Server/1 -> Entity Output Switch/1

== system lib_TerCtrl_MASmsg/MAS messages/ID1/Send to neighbor/five/select ==
  select : TriggerPort  TriggerType=function-call  IsSimulinkFunction=on  FunctionName=select  FunctionVisibility=scoped  VariantControl=(inherit)
  All : simulink/Logic and Bit Operations/Compare To Constant  relop===  const=0  OutDataTypeStr=boolean  ZeroCross=off
  Gain : Gain  OutDataTypeStr=double
  Gain1 : Gain  Gain=2  OutDataTypeStr=double
  Gain2 : Gain  Gain=6  OutDataTypeStr=double
  Gain3 : Gain  Gain=3  OutDataTypeStr=double
  Gain4 : Gain  Gain=4  OutDataTypeStr=double
  Gain5 : Gain  Gain=5  OutDataTypeStr=double
  Neighbor1 : simulink/Logic and Bit Operations/Compare To Constant  relop===  const=2  OutDataTypeStr=boolean  ZeroCross=off
  Neighbor2 : simulink/Logic and Bit Operations/Compare To Constant  relop===  const=2  OutDataTypeStr=boolean  ZeroCross=off
  Neighbor3 : simulink/Logic and Bit Operations/Compare To Constant  relop===  const=0  OutDataTypeStr=boolean  ZeroCross=off
  Neighbor4 : simulink/Logic and Bit Operations/Compare To Constant  relop===  const=0  OutDataTypeStr=boolean  ZeroCross=off
  Neighbor5 : simulink/Logic and Bit Operations/Compare To Constant  relop===  const=0  OutDataTypeStr=boolean  ZeroCross=off
  Sum : Sum  Inputs=|++++++
  u : ArgIn  DisableCoverage=on  ArgumentName=u
  y : ArgOut  ArgumentName=y
  wires:
  Neighbor5/1 -> Gain5/1
  Gain5/1 -> Sum/5
  Neighbor2/1 -> Gain1/1
  u/1 -> Neighbor3/1, Neighbor4/1, All/1, Neighbor5/1, Neighbor1/1, Neighbor2/1
  Neighbor1/1 -> Gain/1
  Gain2/1 -> Sum/6
  All/1 -> Gain2/1
  Gain1/1 -> Sum/2
  Sum/1 -> y/1
  Gain/1 -> Sum/1
  Neighbor3/1 -> Gain3/1
  Gain3/1 -> Sum/3
  Gain4/1 -> Sum/4
  Neighbor4/1 -> Gain4/1

== system lib_TerCtrl_MASmsg/MAS messages/ID1/Send to neighbor/four/select ==
  select : TriggerPort  TriggerType=function-call  IsSimulinkFunction=on  FunctionName=select  FunctionVisibility=scoped  VariantControl=(inherit)
  All : simulink/Logic and Bit Operations/Compare To Constant  relop===  const=0  OutDataTypeStr=boolean  ZeroCross=off
  Gain : Gain  OutDataTypeStr=double
  Gain1 : Gain  Gain=2  OutDataTypeStr=double
  Gain2 : Gain  Gain=5  OutDataTypeStr=double
  Gain3 : Gain  Gain=3  OutDataTypeStr=double
  Gain4 : Gain  Gain=4  OutDataTypeStr=double
  Neighbor1 : simulink/Logic and Bit Operations/Compare To Constant  relop===  const=1  OutDataTypeStr=boolean  ZeroCross=off
  Neighbor2 : simulink/Logic and Bit Operations/Compare To Constant  relop===  const=3  OutDataTypeStr=boolean  ZeroCross=off
  Neighbor3 : simulink/Logic and Bit Operations/Compare To Constant  relop===  const=0  OutDataTypeStr=boolean  ZeroCross=off
  Neighbor4 : simulink/Logic and Bit Operations/Compare To Constant  relop===  const=0  OutDataTypeStr=boolean  ZeroCross=off
  Sum : Sum  Inputs=|+++++
  u : ArgIn  DisableCoverage=on  ArgumentName=u
  y : ArgOut  ArgumentName=y
  wires:
  Neighbor4/1 -> Gain4/1
  Gain4/1 -> Sum/4
  Gain3/1 -> Sum/3
  Neighbor3/1 -> Gain3/1
  Gain/1 -> Sum/1
  Sum/1 -> y/1
  Gain1/1 -> Sum/2
  All/1 -> Gain2/1
  Gain2/1 -> Sum/5
  Neighbor1/1 -> Gain/1
  u/1 -> Neighbor2/1, Neighbor1/1, All/1, Neighbor4/1, Neighbor3/1
  Neighbor2/1 -> Gain1/1

== system lib_TerCtrl_MASmsg/MAS messages/ID1/Send to neighbor/one/select ==
  select : TriggerPort  TriggerType=function-call  IsSimulinkFunction=on  FunctionName=select  FunctionVisibility=scoped  VariantControl=(inherit)
  All : simulink/Logic and Bit Operations/Compare To Constant  relop===  const=0  OutDataTypeStr=boolean  ZeroCross=off
  Gain : Gain  OutDataTypeStr=double
  Gain2 : Gain  Gain=2  OutDataTypeStr=double
  Neighbor : simulink/Logic and Bit Operations/Compare To Constant  relop===  const=2  OutDataTypeStr=boolean  ZeroCross=off
  Sum : Sum  Inputs=|++
  u : ArgIn  DisableCoverage=on  ArgumentName=u
  y : ArgOut  ArgumentName=y
  wires:
  Gain/1 -> Sum/1
  Sum/1 -> y/1
  All/1 -> Gain2/1
  Gain2/1 -> Sum/2
  Neighbor/1 -> Gain/1
  u/1 -> Neighbor/1, All/1

== system lib_TerCtrl_MASmsg/MAS messages/ID1/Send to neighbor/three/select ==
  select : TriggerPort  TriggerType=function-call  IsSimulinkFunction=on  FunctionName=select  FunctionVisibility=scoped  VariantControl=(inherit)
  All : simulink/Logic and Bit Operations/Compare To Constant  relop===  const=0  OutDataTypeStr=boolean  ZeroCross=off
  Gain : Gain  OutDataTypeStr=double
  Gain1 : Gain  Gain=2  OutDataTypeStr=double
  Gain2 : Gain  Gain=4  OutDataTypeStr=double
  Gain3 : Gain  Gain=3  OutDataTypeStr=double
  Neighbor1 : simulink/Logic and Bit Operations/Compare To Constant  relop===  const=0  OutDataTypeStr=boolean  ZeroCross=off
  Neighbor2 : simulink/Logic and Bit Operations/Compare To Constant  relop===  const=0  OutDataTypeStr=boolean  ZeroCross=off
  Neighbor3 : simulink/Logic and Bit Operations/Compare To Constant  relop===  const=0  OutDataTypeStr=boolean  ZeroCross=off
  Sum : Sum  Inputs=|++++
  u : ArgIn  DisableCoverage=on  ArgumentName=u
  y : ArgOut  ArgumentName=y
  wires:
  Gain3/1 -> Sum/3
  Neighbor3/1 -> Gain3/1
  Gain/1 -> Sum/1
  Sum/1 -> y/1
  Gain1/1 -> Sum/2
  All/1 -> Gain2/1
  Gain2/1 -> Sum/4
  Neighbor1/1 -> Gain/1
  u/1 -> Neighbor2/1, Neighbor1/1, All/1, Neighbor3/1
  Neighbor2/1 -> Gain1/1

== system lib_TerCtrl_MASmsg/MAS messages/ID1/Send to neighbor/two/select ==
  select : TriggerPort  TriggerType=function-call  IsSimulinkFunction=on  FunctionName=select  FunctionVisibility=scoped  VariantControl=(inherit)
  All : simulink/Logic and Bit Operations/Compare To Constant  relop===  const=0  OutDataTypeStr=boolean  ZeroCross=off
  Gain : Gain  OutDataTypeStr=double
  Gain1 : Gain  Gain=2  OutDataTypeStr=double
  Gain2 : Gain  Gain=3  OutDataTypeStr=double
  Neighbor1 : simulink/Logic and Bit Operations/Compare To Constant  relop===  const=7  OutDataTypeStr=boolean  ZeroCross=off
  Neighbor2 : simulink/Logic and Bit Operations/Compare To Constant  relop===  const=2  OutDataTypeStr=boolean  ZeroCross=off
  Sum : Sum  Inputs=|+++
  u : ArgIn  DisableCoverage=on  ArgumentName=u
  y : ArgOut  ArgumentName=y
  wires:
  Gain/1 -> Sum/1
  Sum/1 -> y/1
  Gain1/1 -> Sum/2
  All/1 -> Gain2/1
  Gain2/1 -> Sum/3
  Neighbor1/1 -> Gain/1
  u/1 -> Neighbor2/1, Neighbor1/1, All/1
  Neighbor2/1 -> Gain1/1

== system lib_TerCtrl_MASmsg/MAS messages/ID1/Send to neighbor1/five/select ==
  select : TriggerPort  TriggerType=function-call  IsSimulinkFunction=on  FunctionName=select  FunctionVisibility=scoped  VariantControl=(inherit)
  All : simulink/Logic and Bit Operations/Compare To Constant  relop===  const=0  OutDataTypeStr=boolean  ZeroCross=off
  Gain : Gain  OutDataTypeStr=double
  Gain1 : Gain  Gain=2  OutDataTypeStr=double
  Gain2 : Gain  Gain=6  OutDataTypeStr=double
  Gain3 : Gain  Gain=3  OutDataTypeStr=double
  Gain4 : Gain  Gain=4  OutDataTypeStr=double
  Gain5 : Gain  Gain=5  OutDataTypeStr=double
  Neighbor1 : simulink/Logic and Bit Operations/Compare To Constant  relop===  const=2  OutDataTypeStr=boolean  ZeroCross=off
  Neighbor2 : simulink/Logic and Bit Operations/Compare To Constant  relop===  const=2  OutDataTypeStr=boolean  ZeroCross=off
  Neighbor3 : simulink/Logic and Bit Operations/Compare To Constant  relop===  const=0  OutDataTypeStr=boolean  ZeroCross=off
  Neighbor4 : simulink/Logic and Bit Operations/Compare To Constant  relop===  const=0  OutDataTypeStr=boolean  ZeroCross=off
  Neighbor5 : simulink/Logic and Bit Operations/Compare To Constant  relop===  const=0  OutDataTypeStr=boolean  ZeroCross=off
  Sum : Sum  Inputs=|++++++
  u : ArgIn  DisableCoverage=on  ArgumentName=u
  y : ArgOut  ArgumentName=y
  wires:
  Neighbor4/1 -> Gain4/1
  Gain4/1 -> Sum/4
  Gain3/1 -> Sum/3
  Neighbor3/1 -> Gain3/1
  Gain/1 -> Sum/1
  Sum/1 -> y/1
  Gain1/1 -> Sum/2
  All/1 -> Gain2/1
  Gain2/1 -> Sum/6
  Neighbor1/1 -> Gain/1
  u/1 -> Neighbor2/1, Neighbor1/1, Neighbor5/1, All/1, Neighbor4/1, Neighbor3/1
  Neighbor2/1 -> Gain1/1
  Gain5/1 -> Sum/5
  Neighbor5/1 -> Gain5/1
